simulink model "Performance_Analysis"  (R2024a)
settings: Solver=VariableStepAuto  StartTime=0.0  StopTime=3600*24*365*3  FixedStep=Ts  MaxStep=Ts  RelTol=1e-4
values from neighbouring files (symbols this model uses):
  eff_cc = 0.95    [Performance_Analysis_Runner.m]
  effConv = sqrt(0.92)    [Performance_Analysis_Runner.m]
  f = 50    [Performance_Analysis_Runner.m]
  Nb_p = 7    [Performance_Analysis_Runner.m]
  Nb_s = 2    [Performance_Analysis_Runner.m]
  Q = 5120    [Performance_Analysis_Runner.m]
  Ts = 3600    [Performance_Analysis_Runner.m]
  V = 400    [Performance_Analysis_Runner.m]
  Vnom = 25.6    [Performance_Analysis_Runner.m]
undefined symbols (not defined in the file or in its folder): Ion, Lithium
libraries: spsACVoltageSourceLib x3, spsThreePhaseDynamicLoadLib x3, spsBatteryLib x1, spsControlledCurrentSourceLib x1, fl_lib x1, spsGroundLib x1, spsThreePhaseVIMeasurementLib x1, spspowerguiLib x1
Description:
  | Copyright 2008-2014 The MathWorks, Inc.
settings Model: Creator=MathWorks  LastModifiedBy=alexn
settings SolverCC: AlgebraicLoopSolver=TrustRegion
settings DataIOCC: SaveFormat=Array  SignalLoggingSaveFormat=ModelDataLogs  SaveOutput=off  SaveTime=off  ReturnWorkspaceOutputs=off  SignalLoggingName=sigsOut
settings OptimizationCC: BooleanDataType=off  ExpressionDepthLimit=2147483647  InitFltsAndDblsToZero=on  EfficientMapNaN2IntZero=off  LifeSpan=inf
settings DebuggingCC: SaveWithParameterizedLinksMsg=none  UnderspecifiedInitializationDetection=Classic  MergeDetectMultiDrivingBlocksExec=none  CheckExecutionContextPreStartOutputMsg=on  SignalResolutionControl=TryResolveAllWithWarning  MultiTaskDSMMsg=warning  MultiTaskCondExecSysMsg=none  SigSpecEnsureSampleTimeMsg=none  FcnCallInpInsideContextMsg=warning  UnconnectedInputMsg=warning  UnconnectedOutputMsg=warning  UnconnectedLineMsg=warning  StateNameClashWarn=warning  SFUnexpectedBacktrackingDiag=warning  SFNoUnconditionalDefaultTransitionDiag=warning  SFExecutionAtInitializationDiag=none  ArithmeticOperatorsInVariantConditions=warning
settings HardwareCC: ProdBitPerInt=16  ProdBitPerPointer=16  ProdBitPerSizeT=32  ProdBitPerPtrDiffT=32  ProdLargestAtomicFloat=None  ProdIntDivRoundTo=Undefined  ProdEndianess=Unspecified  ProdWordSize=32  ProdHWDeviceType=Specified  TargetUnknown=on
settings ModelReferenceCC: EnableRefExpFcnMdlSchedulingChecks=on  PropagateSignalLabelsOutOfModel=off
settings SFSimCC: SimUseLocalCustomCode=off  CustomCodeUndefinedFunction=UseInterfaceOnly
settings RTWCC: RTWUseLocalCustomCode=off  GPUComputeCapability=3.5  DLArmComputeVersion=19.05
settings CodeAppCC: StateflowObjectComments=on
settings GRTTargetCC: TargetFcnLib=ansi_tfl_tmw.mat  TargetLangStandard=C89/C90 (ANSI)  CombineOutputUpdateFcns=off  GRTInterface=on
settings ConfigComp: CovMetricSettings=dw  CovSaveCumulativeToWorkspaceVar=on  CovSaveSingleToWorkspaceVar=on  CovExternalEMLEnable=off  CovSFcnEnable=off
settings SimscapeCC: SimscapeNormalizeSystem=off

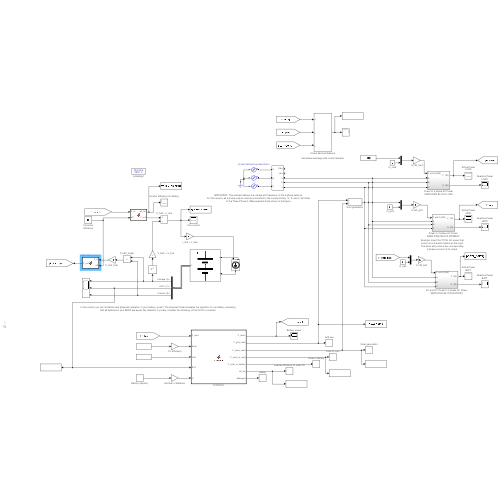
[thumbnail: Simulink's stored preview of the top-level diagram]
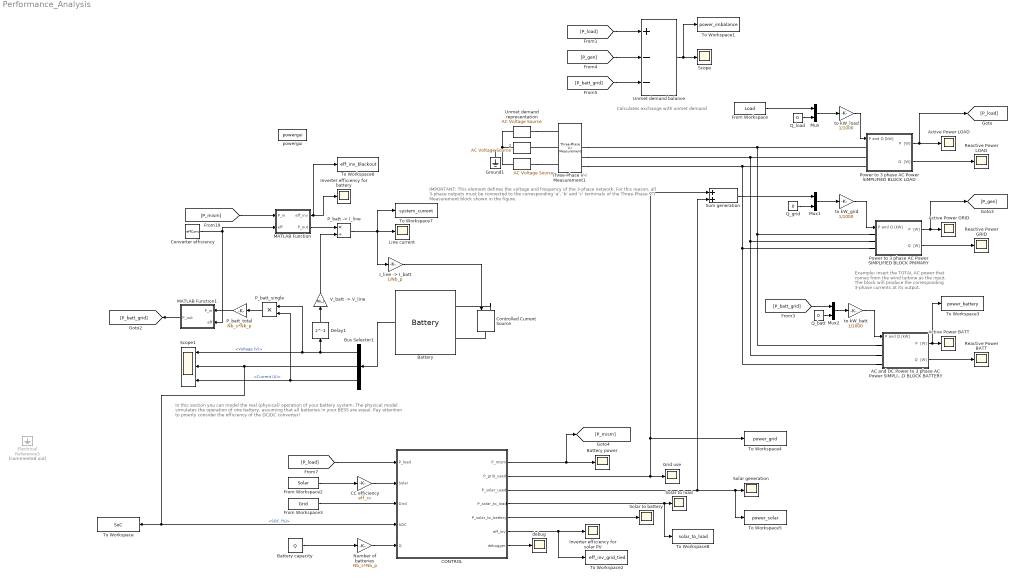
== system Performance_Analysis ==
  note: IMPORTANT: This element defines the voltage and frequency of the 3-phase network.
      | For this reason, all 3-phase outputs must be connected to the corresponding  'a', 'b' and 'c' terminals
      | of the Three-Phase V-I Measurement block shown in the figure.
  note: Example: insert the TOTAL AC power that
      | comes from the wind turbine as the input.
      | The block will produce the corresponding
      | 3-phase currents at its output.
  note: In this section you can model the real (physical) operation of your battery system. The physical model simulates the operation of one battery, assuming that all batteries in your BESS are equal. Pay attention to proerly consider the efficiency of the DC/DC converter!
  note: Calculates exchange with unmet demand
  " " : spsACVoltageSourceLib/AC Voltage Source  Amplitude=V*sqrt(3)  Phase=-240  Frequency=f  SampleTime=-1  Measurements=None  BusType=swing  Pref=10e3  Qref=0  Qmin=-inf  Qmax=+inf
  "    1" : spsACVoltageSourceLib/AC Voltage Source  Amplitude=V*sqrt(3)  Phase=-120  Frequency=f  SampleTime=-1  Measurements=None  BusType=swing  Pref=10e3  Qref=0  Qmin=-inf  Qmax=+inf
  AC and DC Power to 3 phase AC Power SIMPLIFIED BLOCK BATTERY : Subsystem
  Active Power BATT : Scope
  Active Power GRID : Scope
  Active Power LOAD : Scope
  Battery : spsBatteryLib/Battery  BatType=Lithium-Ion  ShowTempParam=off  ThermalPreset=no  ShowAgeParam=on  NomV=Vnom  NomQ=AH  SOC=SOC0  Batt_Tr=0.1  PresetModel=on  MaxQ=200  MinV=19.2  FullV=29.7981  Dis_rate=86.9565  R=0.00128  Normal_OP=180.8696  expZone="[27.6579      9.82609]"  current=15  Units=Ampere-hour  Tci=20  NomT=25  T2=0  MaxQ2=2.208  FullV2=3.45  Normal_OP2=2.8  expZone2="[3.22        0.23]"  Rca=0.6  ti=1000  Dp=0  Neq0=0  Tsim=3600  Ta1=25  Qeol=AH_EOL  Reol=0.013333*1.2  Char_age=[2.3478, 3]  Dis_age=[2.3478, 10]  N1=1500  N2=10500  N3=1000  N4=1400  Ta2=45  N5=950
      link override Model/Saturation: UpperLimit=95  LowerLimit=5
  Battery capacity : Constant  Value=Q
  Battery power : Scope
  Bus Selector1 : BusSelector  OutputSignals=Voltage (V),SOC (%),Current (A)
  CC efficiency : Gain  Gain=eff_cc
  CONTROL : MATLAB Function  TreatAsAtomicUnit=on
  Controlled Current Source : spsControlledCurrentSourceLib/Controlled Current Source  Initialize=on  Source_Type=AC  Amplitude=0  Phase=0  Frequency=0  Measurements=None
  Converter efficiency : Constant  Value=effConv
  Delay1 : Delay  DelayLength=1  InitialCondition=Vnom
  Electrical Reference3 : fl_lib/Electrical/Electrical Elements/Electrical Reference  Commented=on
  From Workspace : FromWorkspace  VariableName=Load  SampleTime=-1
  From Workspace2 : FromWorkspace  VariableName=Solar  SampleTime=-1
  From Workspace3 : FromWorkspace  VariableName=Grid  SampleTime=-1
  Grid use : Scope
  Ground1 : spsGroundLib/Ground  LConnTagsString=a
  "I_line -> I_batt " : Gain  Gain=1/Nb_p
  Inverter efficiency for battery : Scope
  Inverter efficiency for solar PV : Scope
  Line current : Scope
  MATLAB Function : MATLAB Function  TreatAsAtomicUnit=on
  MATLAB Function1 : MATLAB Function  TreatAsAtomicUnit=on
  Mux : Mux  Inputs=2
  Mux1 : Mux  Inputs=2
  Mux2 : Mux  Inputs=2
  Number of batteries : Gain  Gain=Nb_s*Nb_p
  "P_batt -> I_line" : Product  Inputs=*/
  P_batt_single : Product  Inputs=**
  P_batt_total : Gain  Gain=Nb_s*Nb_p
  Power to 3 phase AC Power SIMPLIFIED BLOCK LOAD : Subsystem
  Power to 3 phase AC Power SIMPLIFIED BLOCK PRIMARY : Subsystem
  Q_batt : Constant  Value=0
  Q_grid : Constant  Value=0
  Q_load : Constant  Value=0
  Reactive Power BATT : Scope
  Reactive Power GRID : Scope
  Reactive Power LOAD : Scope
  Scope : Scope
  Scope1 : Scope  NumInputPorts=3
  Solar generation : Scope
  Solar to battery : Scope
  Solar to load : Scope
  Sum generation : Sum
  Three-Phase V-I Measurement1 : spsThreePhaseVIMeasurementLib/Three-Phase V-I Measurement  VoltageMeasurement=phase-to-phase  SetLabelV=off  LabelV=Vabc  Vpu=off  VpuLL=off  CurrentMeasurement=yes  SetLabelI=off  LabelI=Iabc  Ipu=off  Pbase=100e6  Vbase=500e3  OutputType=Complex  PhasorSimulation=off  PSBequivalent=0
  To Workspace : ToWorkspace  VariableName=SoC  SampleTime=-1
  To Workspace1 : ToWorkspace  VariableName=power_imbalance  SaveFormat=Timeseries  SampleTime=-1
  To Workspace2 : ToWorkspace  VariableName=eff_inv_grid_tied  SaveFormat=Timeseries  SampleTime=-1
  To Workspace3 : ToWorkspace  VariableName=power_battery  SaveFormat=Timeseries  SampleTime=-1
  To Workspace4 : ToWorkspace  VariableName=power_grid  SaveFormat=Timeseries  SampleTime=-1
  To Workspace5 : ToWorkspace  VariableName=power_solar  SaveFormat=Timeseries  SampleTime=-1
  To Workspace6 : ToWorkspace  VariableName=eff_inv_blackout  SaveFormat=Timeseries  SampleTime=-1
  To Workspace7 : ToWorkspace  VariableName=system_current  SaveFormat=Timeseries  SampleTime=-1
  To Workspace8 : ToWorkspace  VariableName=solar_to_load  SaveFormat=Timeseries  SampleTime=-1
  Unmet demand balance : Sum  Inputs=+--
  Unmet demand representation : spsACVoltageSourceLib/AC Voltage Source  Amplitude=V*sqrt(3)  Phase=0  Frequency=f  SampleTime=-1  Measurements=None  BusType=swing  Pref=10e3  Qref=0  Qmin=-inf  Qmax=+inf
  "V_batt -> V_line" : Gain  Gain=Nb_s
  debug : Scope
  powergui : spspowerguiLib/powergui  SimulationMode=Discrete  SampleTime=Ts  frequency=60  Iterations=50  frequencyindice=50  Pbase=100e6  ErrMax=1e-4  UnitsV=kV  UnitsW=MW  buscounter=0  FunctionMessages=off  echomessages=off  EnableUseOfTLC=off  CurrentSourceSwitches=off  DisableSnubberDevices=off  DisableRonSwitches=off  DisableVfSwitches=off  DisplayEquations=off  AutomaticDiscreteSolvers=off  SolverType=Tustin/Backward Euler (TBE)  Interpol=off  ExternalGateDelay=off  methode=off  Ts=0  x0status=blocks  SPID=off  SwTol=0  HookPort=off  NonlinearTolerance=1e-4  nMaxIteration=100  ContinueOnMaxIteration=off  RestoreLinks=warning  ResistiveCurrentMeasurement=off  Frange=[0:2:500]  Ylog=off  Xlog=on  ShowGrid=off  save=off  variable=ZData  structure=0  ZoomFFT=on  StartTime=0.0  cycles=1  DisplayStyle=1  fundamental=60  FreqAxis=off  MaxFrequency=1000  frequencyindicesteady=1  RmsSteady=1  display=off
  to kW_batt : Gain  Gain=1/1000
  to kW_grid : Gain  Gain=1/1000
  to kW_load : Gain  Gain=1/1000
  wires:
  Q_load/1 -> Mux/2
  Mux/1 -> to kW_load/1
  Power to 3 phase AC Power SIMPLIFIED BLOCK LOAD/1("P  [W] ") -> [P_load], Active Power LOAD/1
  Power to 3 phase AC Power SIMPLIFIED BLOCK LOAD/2("Q  [W] ") -> Reactive Power LOAD/1
  Q_grid/1 -> Mux1/2
  Power to 3 phase AC Power SIMPLIFIED BLOCK PRIMARY/1("P  [W] ") -> [P_gen], Active Power GRID/1
  Sum generation/1 -> Mux1/1
  Mux1/1 -> to kW_grid/1
  to kW_grid/1 -> Power to 3 phase AC Power SIMPLIFIED BLOCK PRIMARY/1(P and Q [kW])
  Q_batt/1 -> Mux2/2
  to kW_batt/1 -> AC and DC Power to 3 phase AC Power SIMPLIFIED BLOCK BATTERY/1(P and Q [kW])
  Mux2/1 -> to kW_batt/1
  to kW_load/1 -> Power to 3 phase AC Power SIMPLIFIED BLOCK LOAD/1(P and Q [kW])
  Power to 3 phase AC Power SIMPLIFIED BLOCK PRIMARY/2("Q  [W] ") -> Reactive Power GRID/1
  AC and DC Power to 3 phase AC Power SIMPLIFIED BLOCK BATTERY/1("P  [W] ") -> To Workspace3/1, Active Power BATT/1
  AC and DC Power to 3 phase AC Power SIMPLIFIED BLOCK BATTERY/2("Q  [W] ") -> Reactive Power BATT/1
  Battery/1 -> Bus Selector1/1
  Bus Selector1/1 -> P_batt_single/1, Scope1/1, Delay1/1  "<Voltage (V)>"
  "V_batt -> V_line"/1 -> "P_batt -> I_line"/2
  Delay1/1 -> "V_batt -> V_line"/1
  "P_batt -> I_line"/1 -> To Workspace7/1, "I_line -> I_batt "/1, Line current/1
  "I_line -> I_batt "/1 -> Controlled Current Source/1
  Bus Selector1/2 -> To Workspace/1, CONTROL/4(SOC), Scope1/2  "<SOC (%)>"
  Bus Selector1/3 -> P_batt_single/2, Scope1/3  "<Current (A)>"
  P_batt_single/1 -> P_batt_total/1
  P_batt_total/1 -> MATLAB Function1/1(P_in)
  [P_mism] -> MATLAB Function/1(P_in)
  MATLAB Function/2(P_out) -> "P_batt -> I_line"/1
  MATLAB Function1/1(P_out) -> [P_batt_grid]
  Converter efficiency/1 -> MATLAB Function1/2(eff), MATLAB Function/2(eff)
  From Workspace/1 -> Mux/1
  [P_batt_grid] -> Unmet demand balance/3
  [P_gen] -> Unmet demand balance/2
  Unmet demand balance/1 -> To Workspace1/1, Scope/1
  [P_load] -> Unmet demand balance/1
  [P_load] -> CONTROL/1(P_load)
  CONTROL/1(P_mism) -> [P_mism], Battery power/1
  From Workspace2/1 -> CC efficiency/1
  CONTROL/3(P_solar_used) -> To Workspace5/1, Solar generation/1, Sum generation/2
  CONTROL/4(P_solar_to_load) -> To Workspace8/1, Solar to load/1
  CONTROL/5(P_solar_to_battery) -> Solar to battery/1
  Battery capacity/1 -> Number of batteries/1
  Number of batteries/1 -> CONTROL/5(Q)
  From Workspace3/1 -> CONTROL/3(Grid)
  CC efficiency/1 -> CONTROL/2(Solar)
  CONTROL/6(eff_inv) -> Inverter efficiency for solar PV/1, To Workspace2/1
  CONTROL/7(debugger) -> debug/1
  [P_batt_grid] -> Mux2/1
  MATLAB Function/1(eff_inv) -> To Workspace6/1, Inverter efficiency for battery/1
  CONTROL/2(P_grid_used) -> Grid use/1, To Workspace4/1, Sum generation/1
  connections:
  Ground1/LConn1 -- "    1"/LConn1 -- Unmet demand representation/LConn1 -- " "/LConn1
  " "/RConn1 -- Three-Phase V-I Measurement1/LConn3
  Three-Phase V-I Measurement1/LConn2 -- "    1"/RConn1
  Unmet demand representation/RConn1 -- Three-Phase V-I Measurement1/LConn1
  Three-Phase V-I Measurement1/RConn2 -- AC and DC Power to 3 phase AC Power SIMPLIFIED BLOCK BATTERY/LConn2 -- Power to 3 phase AC Power SIMPLIFIED BLOCK PRIMARY/LConn2 -- Power to 3 phase AC Power SIMPLIFIED BLOCK LOAD/LConn2
  Three-Phase V-I Measurement1/RConn3 -- Power to 3 phase AC Power SIMPLIFIED BLOCK LOAD/LConn3 -- AC and DC Power to 3 phase AC Power SIMPLIFIED BLOCK BATTERY/LConn3 -- Power to 3 phase AC Power SIMPLIFIED BLOCK PRIMARY/LConn3
  Three-Phase V-I Measurement1/RConn1 -- AC and DC Power to 3 phase AC Power SIMPLIFIED BLOCK BATTERY/LConn1 -- Power to 3 phase AC Power SIMPLIFIED BLOCK PRIMARY/LConn1 -- Power to 3 phase AC Power SIMPLIFIED BLOCK LOAD/LConn1
  Controlled Current Source/LConn1 -- Battery/LConn1
  Controlled Current Source/RConn1 -- Battery/LConn2

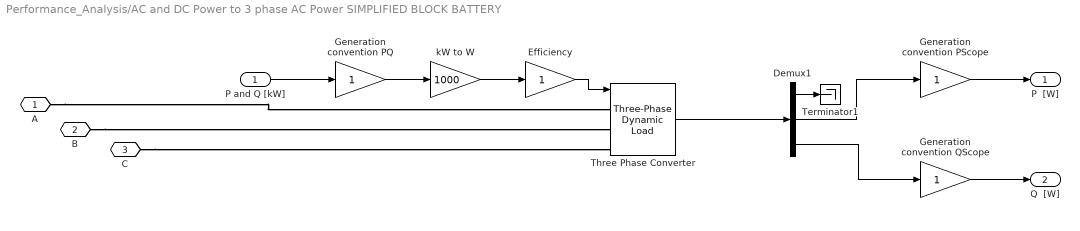
== system Performance_Analysis/AC and DC Power to 3 phase AC Power SIMPLIFIED BLOCK BATTERY ==
  P and Q [kW] : Inport
  Demux1 : Demux  Outputs=3
      settings: DisplayOption=none
  Efficiency : Gain
  Generation convention PQ : Gain
  Generation convention PScope : Gain
  Generation convention QScope : Gain
  Terminator1 : Terminator
  Three Phase Converter : spsThreePhaseDynamicLoadLib/Three-Phase Dynamic Load  NominalVoltage=[ V/sqrt(3) f ]  ActiveReactivePowers=[1e+003 0]  PositiveSequence=[0.98441 -1.41063]  ExternalControl=on  NpNq="[1  1]"  TimeConstants="[0  0  0  0]"  MinimumVoltage=0.7  Tfilter=1e-4  LoadFlowParameters=[4 50000000 0 0 25000000]
  kW to W : Gain  Gain=1000
  A : PMIOPort  Side=Left
  B : PMIOPort  Port=2  Side=Left
  C : PMIOPort  Port=3  Side=Left
  "P  [W] " : Outport
  "Q  [W] " : Outport  Port=2
  wires:
  Demux1/1 -> Terminator1/1
  Three Phase Converter/1 -> Demux1/1
  Efficiency/1 -> Three Phase Converter/1
  kW to W/1 -> Efficiency/1
  Generation convention PQ/1 -> kW to W/1
  P and Q [kW]/1 -> Generation convention PQ/1
  Generation convention PScope/1 -> "P  [W] "/1
  Demux1/2 -> Generation convention PScope/1
  Demux1/3 -> Generation convention QScope/1
  Generation convention QScope/1 -> "Q  [W] "/1
  connections:
  A/RConn1 -- Three Phase Converter/LConn1
  C/RConn1 -- Three Phase Converter/LConn3
  B/RConn1 -- Three Phase Converter/LConn2

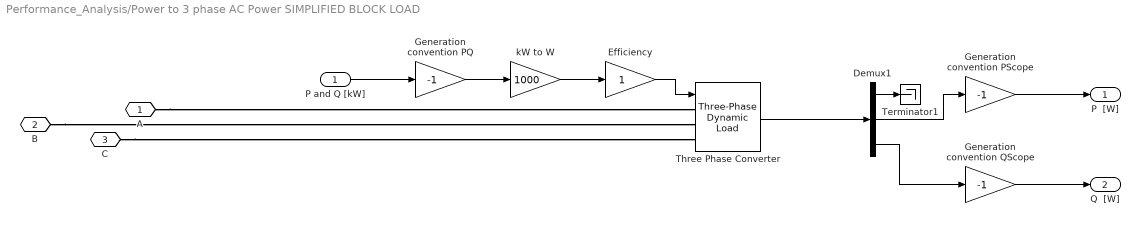
== system Performance_Analysis/Power to 3 phase AC Power SIMPLIFIED BLOCK LOAD ==
  P and Q [kW] : Inport
  Demux1 : Demux  Outputs=3
      settings: DisplayOption=none
  Efficiency : Gain
  Generation convention PQ : Gain  Gain=-1
  Generation convention PScope : Gain  Gain=-1
  Generation convention QScope : Gain  Gain=-1
  Terminator1 : Terminator
  Three Phase Converter : spsThreePhaseDynamicLoadLib/Three-Phase Dynamic Load  NominalVoltage=[ V/sqrt(3) f ]  ActiveReactivePowers=[1000 0]  PositiveSequence=[0.98441 -1.41063]  ExternalControl=on  NpNq="[1  1]"  TimeConstants="[0  0  0  0]"  MinimumVoltage=0.7  Tfilter=1e-4  LoadFlowParameters=[4 50000000 0 0 25000000]
  kW to W : Gain  Gain=1000
  A : PMIOPort  Side=Left
  B : PMIOPort  Port=2  Side=Left
  C : PMIOPort  Port=3  Side=Left
  "P  [W] " : Outport
  "Q  [W] " : Outport  Port=2
  wires:
  Demux1/1 -> Terminator1/1
  Efficiency/1 -> Three Phase Converter/1
  kW to W/1 -> Efficiency/1
  Generation convention PQ/1 -> kW to W/1
  P and Q [kW]/1 -> Generation convention PQ/1
  Generation convention PScope/1 -> "P  [W] "/1
  Demux1/2 -> Generation convention PScope/1
  Demux1/3 -> Generation convention QScope/1
  Generation convention QScope/1 -> "Q  [W] "/1
  Three Phase Converter/1 -> Demux1/1
  connections:
  A/RConn1 -- Three Phase Converter/LConn1
  C/RConn1 -- Three Phase Converter/LConn3
  B/RConn1 -- Three Phase Converter/LConn2

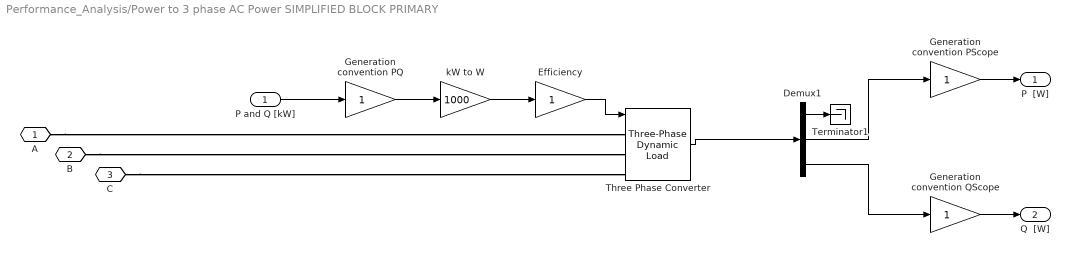
== system Performance_Analysis/Power to 3 phase AC Power SIMPLIFIED BLOCK PRIMARY ==
  P and Q [kW] : Inport
  Demux1 : Demux  Outputs=3
      settings: DisplayOption=none
  Efficiency : Gain
  Generation convention PQ : Gain
  Generation convention PScope : Gain
  Generation convention QScope : Gain
  Terminator1 : Terminator
  Three Phase Converter : spsThreePhaseDynamicLoadLib/Three-Phase Dynamic Load  NominalVoltage=[ V/sqrt(3) f ]  ActiveReactivePowers=[1e+003 0]  PositiveSequence=[0.98441 -1.41063]  ExternalControl=on  NpNq="[1  1]"  TimeConstants="[0  0  0  0]"  MinimumVoltage=0.7  Tfilter=1e-4  LoadFlowParameters=[4 50000000 0 0 25000000]
  kW to W : Gain  Gain=1000
  A : PMIOPort  Side=Left
  B : PMIOPort  Port=2  Side=Left
  C : PMIOPort  Port=3  Side=Left
  "P  [W] " : Outport
  "Q  [W] " : Outport  Port=2
  wires:
  Demux1/1 -> Terminator1/1
  Three Phase Converter/1 -> Demux1/1
  Efficiency/1 -> Three Phase Converter/1
  kW to W/1 -> Efficiency/1
  Generation convention PQ/1 -> kW to W/1
  P and Q [kW]/1 -> Generation convention PQ/1
  Generation convention PScope/1 -> "P  [W] "/1
  Demux1/2 -> Generation convention PScope/1
  Demux1/3 -> Generation convention QScope/1
  Generation convention QScope/1 -> "Q  [W] "/1
  connections:
  A/RConn1 -- Three Phase Converter/LConn1
  C/RConn1 -- Three Phase Converter/LConn3
  B/RConn1 -- Three Phase Converter/LConn2

== matlab function Performance_Analysis/MATLAB Function1 ==
  data: P_in input; P_out output; eff input
%% Model of BESS power converter

function P_out = fcn(P_in,eff)

if P_in<0
    P_out = P_in/eff/0.98; % Output power calculation
else
    P_out= P_in*eff;
    A = 6.75776E+03;
    B = 4.2E+01;
    C = -1.2E-05;		
    P_ac0 = 6.12E+03;

    P_out = max((((P_ac0/(A-B))-C*(A-B))*(P_out-B)+C*power((P_out-B),2)),0);
end

% Modify this expression to correctly account for the power converter efficiency when charging and discharging!

== matlab function Performance_Analysis/MATLAB Function ==
  data: eff_inv output; P_in input; P_out output; eff input
%% Model of BESS power converter

function [eff_inv, P_out] = fcn(P_in,eff)

eff_inv=0;

if P_in<0
    P_out = 0.98*eff* P_in; % Output power calculation
else
    P_out_0 = P_in/eff;
    A = 6.75776E+03;
    B = 4.2E+01;
    C = -1.2E-05;		
    P_ac0 = 6.12E+03;

    % SNL inverter model inversion
    alpha = C;
    beta = (P_ac0 / (A - B)) - C * (A - B);

    a = alpha;
    b = beta - 2 * alpha * B;
    c = alpha * B^2 - beta * B;

    discriminant = b^2 - 4 * a * (c - P_out_0);
    P_out = max((-b + sqrt(discriminant)) / (2 * a), 0);
    eff_inv=P_out_0/P_out;
end
% Modify this expression to correctly account for the power converter efficiency when charging and discharging!

== matlab function Performance_Analysis/CONTROL ==
  data: P_load input; P_mism output; Solar input; Grid input; P_grid_used output; P_solar_used output; SOC input; P_solar_to_load output; P_solar_to_battery output; Q input; eff_inv output; debugger output
%% Controller model

function [P_mism, P_grid_used, P_solar_used, P_solar_to_load, P_solar_to_battery, eff_inv, debugger] = CONTROL(P_load, Solar, Grid, SOC, Q)
    P_solar_used = Solar;

    P_nom = 6800;
    A = 6.75776E+03;
    B = 4.2E+01;
    C = -1.2E-05;		
    P_ac0 = 6.12E+03;
    eff_inv = 0;
    debugger = 0;


    if Grid == 0 % if blackout, use battery
        if SOC - (P_load/Q)*100 > 15 % if SOC is above 15%, you have battery available
            P_mism = P_load;            
        else % if not, you're cooked
            P_mism=0;
        end
        P_grid_used = Grid;
        P_solar_to_load = 0;
        P_solar_to_battery = 0;
    else % if not blackout, use solar and grid
        if SOC < 95 % if battery is not sufficiently charged, use solar to charge and grid to meet load
            P_mism = -Solar;
            P_grid_used = Grid;
            P_solar_to_load = 0;
            P_solar_to_battery = Solar;
            P_solar_used = Solar;
        else % if battery is charged, use solar to meet load and reduce grid
            Solar_AC = max((((P_ac0/(A-B))-C*(A-B))*(Solar-B)+C*power((Solar-B),2)),0);
            eff_inv = max(Solar_AC/Solar, 0);
            P_mism = 0;
            P_grid_used = P_load - Solar_AC;
            P_solar_to_load = Solar_AC;
            P_solar_to_battery = 0;
            P_solar_used = Solar_AC;
        end
    end
end
